simulink model "HRTIM_main"  (R2023b)
settings: Solver=ode3  StartTime=0.0  StopTime=120e-6  RelTol=1e-3
undefined symbols (not defined in the file): HRTIM_SETB1R_REG_VAL, HRTIM_SETB2R_REG_VAL, HRTIM_SETC1R_REG_VAL, HRTIM_SETC2R_REG_VAL, HRTIM_SL
libraries: dspswit3 x8, simulink x6, simulink_extras x4, hdlsllib x4
(part 2 of 2)

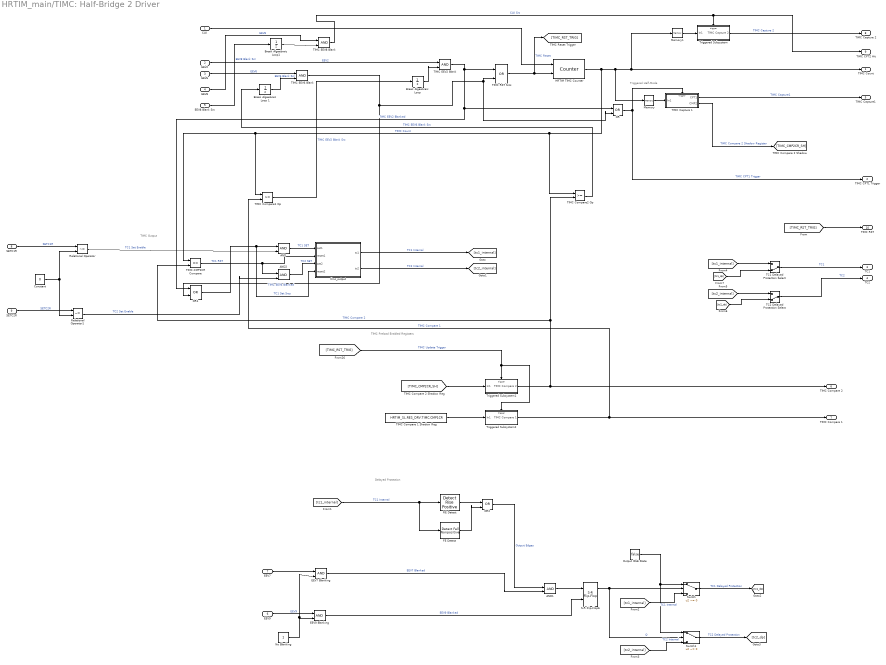
== system HRTIM_main/TIMC: Half-Bridge 2 Driver ==
  note: TIMC Preload Enabled Registers
  note: Triggered Half-Mode
  note: TIMC Output
  note: Delayed Protection
  CLK : Inport
  EEV2 : Inport  Port=2
  EEV6 : Inport  Port=3
  EEV8 : Inport  Port=4
  EEV8 Blank Src : Inport  Port=5
  EEV9 : Inport  Port=6
  EEV7 : Inport  Port=7
  SETC1R : Inport  Port=8
  SETC2R : Inport  Port=9
  AND : Logic  IconShape=distinctive  AllPortsSameDT=off  OutDataTypeStr=boolean
  AND1 : Logic  IconShape=distinctive  AllPortsSameDT=off  OutDataTypeStr=boolean
  AND2 : Logic  IconShape=distinctive  AllPortsSameDT=off  OutDataTypeStr=boolean
  Break Algaebraic Loop : UnitDelay  SampleTime=-1  HasFrameUpgradeWarning=on
  Break Algaebraic Loop 1 : UnitDelay  SampleTime=-1  HasFrameUpgradeWarning=on
  Break Algaebraic Loop1 : UnitDelay  SampleTime=-1  HasFrameUpgradeWarning=on
  Constant : Constant  Value=0  OutDataTypeStr=uint32
  EEV7 Blanking : Logic  IconShape=distinctive  AllPortsSameDT=off  OutDataTypeStr=boolean
  EEV9 Blanking : Logic  IconShape=distinctive  AllPortsSameDT=off  OutDataTypeStr=boolean
  FE Detect : simulink/Logic and Bit Operations/Detect Fall Nonpositive  vinit=0  OutDataTypeStr=boolean
  HRTIM TIMC Counter : dspswit3/Counter  Direction=Up  CountEvent=Rising edge  CounterSize=16 bits  MaxCount=HRTIM_SL.HRTIM_TIMx_FS  InitialCount=0  Output=Count  HitValue=32  ResetInput=on  SamplesPerFrame=1  Ts=1  CntDtype=uint16  HitDtype=Logical
  Memory : Memory  InheritSampleTime=on
  Memory1 : Memory
  No Blanking : Constant
  OR : Logic  Operator=OR  IconShape=distinctive  AllPortsSameDT=off  OutDataTypeStr=boolean
  OR1 : Logic  Operator=OR  IconShape=distinctive  AllPortsSameDT=off  OutDataTypeStr=boolean
  OR2 : Logic  Operator=OR  IconShape=distinctive  AllPortsSameDT=off  OutDataTypeStr=boolean
  Output IDLE State : Constant  Value=false  OutDataTypeStr=boolean
  RE Detect : hdlsllib/Logic and Bit Operations/Detect Rise Positive  vinit=0  OutDataTypeStr=boolean
  Relational Operator : RelationalOperator  Operator=~=  OutDataTypeStr=boolean  RndMeth=Simplest  InputSameDT=off
  Relational Operator1 : RelationalOperator  Operator=~=  OutDataTypeStr=boolean  RndMeth=Simplest  InputSameDT=off
  S-R Flip-Flop6 : simulink_extras/Flip Flops/S-R Flip-Flop  initial_condition=0
  Switch : Switch  Criteria=u2 ~= 0  SaturateOnIntegerOverflow=off  InputSameDT=off
  Switch1 : Switch  Criteria=u2 ~= 0  SaturateOnIntegerOverflow=off  InputSameDT=off
  TC1 Delayed Protection Select : ManualSwitch  CurrentSetting=0
  TC2 Delayed Protection Select : ManualSwitch  CurrentSetting=0
  TIMC Capture 1 : Subsystem  TreatAsAtomicUnit=on
  TIMC Compare 1 Shadow Reg : Constant  Value=HRTIM_SL.RES_DRV.TIMC.CMP1CR
  TIMC Compare1 Op : RelationalOperator  OutDataTypeStr=boolean  RndMeth=Simplest  InputSameDT=off
  TIMC Compare2 Op : RelationalOperator  OutDataTypeStr=boolean  RndMeth=Simplest  InputSameDT=off
  TIMC EEV2 Blank : Logic  IconShape=distinctive  AllPortsSameDT=off  OutDataTypeStr=boolean
  TIMC EEV6 Blank : Logic  IconShape=distinctive  AllPortsSameDT=off  OutDataTypeStr=boolean
  TIMC EEV8 Blank : Logic  IconShape=distinctive  AllPortsSameDT=off  OutDataTypeStr=boolean
  TIMC RST Srcs : Logic  Operator=OR  IconShape=distinctive  AllPortsSameDT=off  OutDataTypeStr=boolean
  TIMC.CMP2CR Compare : RelationalOperator  Operator===  OutDataTypeStr=boolean  RndMeth=Simplest  InputSameDT=off
  Triggered Subsystem : Subsystem  TreatAsAtomicUnit=on
  Triggered Subsystem1 : Subsystem  TreatAsAtomicUnit=on
  Triggered Subsystem2 : Subsystem  TreatAsAtomicUnit=on
  timc_output : MATLAB Function  TreatAsAtomicUnit=on
  TIMC Count : Outport
  TIMC CPT1 Trigger : Outport  Port=2
  TC1 : Outport  Port=3
  TC2 : Outport  Port=4
  TIMC Capture1 : Outport  Port=5
  TIMC Compare 2 : Outport  Port=6
  TIMC Compare 1 : Outport  Port=7
  TIMC Capture 2 : Outport  Port=8
  TIMC CPT2 Hit : Outport  Port=9
  TIMC RST : Outport  Port=10
  wires:
  TIMC EEV6 Blank/1 -> OR1/2, TIMC RST Srcs/2, OR/2  "TIMC EEV6 Blanked"
  [TIMC_CMP2CR_SH] -> Triggered Subsystem1/1(In1)
  HRTIM TIMC Counter/1 -> Memory1/1, TIMC Count/1, Memory/1, TIMC.CMP2CR Compare/1, TIMC Compare1 Op/1, TIMC Compare2 Op/1  "TIMC Count"
  TIMC Compare1 Op/1 -> Break Algaebraic Loop/1  "TIMC EEV2 Blank Src"
  TIMC Capture 1/2(CMP2) -> [TIMC_CMP2CR_SH]  "TIMC Compare 2 Shadow Register"
  TIMC EEV2 Blank/1 -> OR1/1, OR/1, TIMC RST Srcs/1  "TIMC EEV2 Blanked"
  [TIMC_RST_TRIG] -> Triggered Subsystem2/Trigger, Triggered Subsystem1/Trigger  "TIMC Update Trigger"
  TIMC RST Srcs/1 -> HRTIM TIMC Counter/2, [TIMC_RST_TRIG]  "TIMC Reset"
  Memory/1 -> TIMC Capture 1/1(In1)
  Break Algaebraic Loop 1/1 -> TIMC EEV6 Blank/2  "EEV6 Blank Src"
  OR/1 -> TIMC CPT1 Trigger/1, TIMC Capture 1/Trigger  "TIMC CPT1 Trigger"
  Break Algaebraic Loop/1 -> TIMC EEV2 Blank/2
  Triggered Subsystem1/1(TIMC Compare 2) -> TIMC Compare2 Op/2, TIMC.CMP2CR Compare/2, TIMC Compare 2/1  "TIMC Compare 2"
  EEV2/1 -> TIMC EEV2 Blank/1  "EEV2"
  TIMC Compare2 Op/1 -> Break Algaebraic Loop 1/1  "TIMC EEV6 Blank Src"
  Triggered Subsystem2/1(TIMC Compare 1) -> TIMC Compare1 Op/2, TIMC Compare 1/1  "TIMC Compare 1"
  TIMC Compare 1 Shadow Reg/1 -> Triggered Subsystem2/1(In1)
  TIMC Capture 1/1(CPT1) -> TIMC Capture1/1  "TIMC Capture1"
  CLK/1 -> HRTIM TIMC Counter/1
  EEV6/1 -> TIMC EEV6 Blank/1  "EEV6"
  TIMC.CMP2CR Compare/1 -> timc_output/2(reset1), AND2/1  "TC1 RST"
  Triggered Subsystem/1(TIMC Capture 2) -> TIMC Capture 2/1  "TIMC Capture 2"
  EEV8/1 -> TIMC EEV8 Blank/1  "EEV8"
  EEV8 Blank Src/1 -> Break Algaebraic Loop1/1  "EEV8 Blank Src"
  TIMC EEV8 Blank/1 -> Triggered Subsystem/Trigger, TIMC CPT2 Hit/1  "CLK Src"
  Memory1/1 -> Triggered Subsystem/1(In1)
  Break Algaebraic Loop1/1 -> TIMC EEV8 Blank/2
  timc_output/1(tc1) -> [tc1_internal]  "TC1 Internal"
  timc_output/2(tc2) -> [tc2_internal]  "TC2 Internal"
  TC1 Delayed Protection Select/1 -> TC1/1  "TC1"
  [tc1_dp] -> TC1 Delayed Protection Select/2
  [tc2_internal] -> TC2 Delayed Protection Select/1
  [tc2_dp] -> TC2 Delayed Protection Select/2
  TC2 Delayed Protection Select/1 -> TC2/1  "TC2"
  [tc1_internal] -> TC1 Delayed Protection Select/1
  Switch1/1 -> [tc2_dp]  "TC2 Delayed Protection"
  AND1/1 -> S-R Flip-Flop6/1
  [tc2_internal] -> Switch1/3  "TC2 Internal"
  EEV9/1 -> EEV9 Blanking/1  "EEV9"
  [tc1_internal] -> FE Detect/1, RE Detect/1  "TC1 Internal"
  Switch/1 -> [tc1_dp]  "TC1 Delayed Protection"
  RE Detect/1 -> OR2/1
  FE Detect/1 -> OR2/2
  OR2/1 -> AND1/1  "Output Edges"
  EEV7/1 -> EEV7 Blanking/1
  No Blanking/1 -> EEV9 Blanking/2, EEV7 Blanking/2
  EEV7 Blanking/1 -> AND1/2  "EEV7 Blanked"
  [tc1_internal] -> Switch/3  "TC1 Internal"
  S-R Flip-Flop6/1 -> Switch/2, Switch1/2  "Q"
  Output IDLE State/1 -> Switch/1, Switch1/1
  EEV9 Blanking/1 -> S-R Flip-Flop6/2  "EEV9 Blanked"
  [TIMC_RST_TRIG] -> TIMC RST/1
  SETC1R/1 -> Relational Operator/1  "SETC1R"
  Constant/1 -> Relational Operator/2, Relational Operator1/2
  OR1/1 -> AND/1, timc_output/4(reset2)  "TC1 Set Srcs"
  AND/1 -> timc_output/1(set1)  "TC1 SET"
  Relational Operator/1 -> AND/2  "TC1 Set Enable"
  AND2/1 -> timc_output/3(set2)  "TC2 SET"
  Relational Operator1/1 -> AND2/2  "TC2 Set Enable"
  SETC2R/1 -> Relational Operator1/1  "SETC2R"

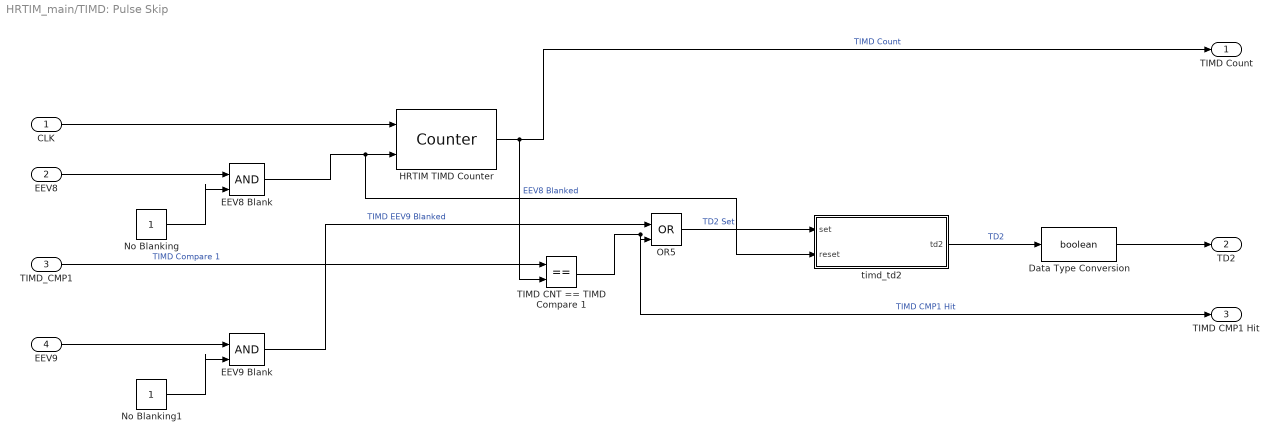
== system HRTIM_main/TIMD: Pulse Skip ==
  CLK : Inport
  EEV8 : Inport  Port=2
  TIMD_CMP1 : Inport  Port=3
  EEV9 : Inport  Port=4
  Data Type Conversion : DataTypeConversion  OutDataTypeStr=boolean  SaturateOnIntegerOverflow=off  RndMeth=Floor
  EEV8 Blank : Logic  IconShape=distinctive  AllPortsSameDT=off  OutDataTypeStr=boolean
  EEV9 Blank : Logic  IconShape=distinctive  AllPortsSameDT=off  OutDataTypeStr=boolean
  HRTIM TIMD Counter : dspswit3/Counter  Direction=Up  CountEvent=Rising edge  CounterSize=16 bits  MaxCount=HRTIM_SL.HRTIM_TIMx_FS  InitialCount=0  Output=Count  HitValue=32  ResetInput=on  SamplesPerFrame=1  Ts=1  CntDtype=uint16  HitDtype=Logical
  No Blanking : Constant
  No Blanking1 : Constant
  OR5 : Logic  Operator=OR  IconShape=distinctive  AllPortsSameDT=off  OutDataTypeStr=boolean
  TIMD CNT == TIMD Compare 1 : RelationalOperator  Operator===  OutDataTypeStr=boolean  RndMeth=Simplest  InputSameDT=off
  timd_td2 : MATLAB Function  TreatAsAtomicUnit=on
  TIMD Count : Outport
  TD2 : Outport  Port=2
  "TIMD CMP1 Hit " : Outport  Port=3
  wires:
  No Blanking/1 -> EEV8 Blank/2
  HRTIM TIMD Counter/1 -> TIMD Count/1, TIMD CNT == TIMD Compare 1/2  "TIMD Count"
  EEV9/1 -> EEV9 Blank/1
  timd_td2/1(td2) -> Data Type Conversion/1  "TD2"
  No Blanking1/1 -> EEV9 Blank/2
  EEV8 Blank/1 -> HRTIM TIMD Counter/2, timd_td2/2(reset)  "EEV8 Blanked"
  TIMD CNT == TIMD Compare 1/1 -> "TIMD CMP1 Hit "/1, OR5/2  "TIMD CMP1 Hit"
  OR5/1 -> timd_td2/1(set)  "TD2 Set"
  CLK/1 -> HRTIM TIMD Counter/1
  EEV9 Blank/1 -> OR5/1  "TIMD EEV9 Blanked"
  EEV8/1 -> EEV8 Blank/1
  TIMD_CMP1/1 -> TIMD CNT == TIMD Compare 1/1  "TIMD Compare 1"
  Data Type Conversion/1 -> TD2/1

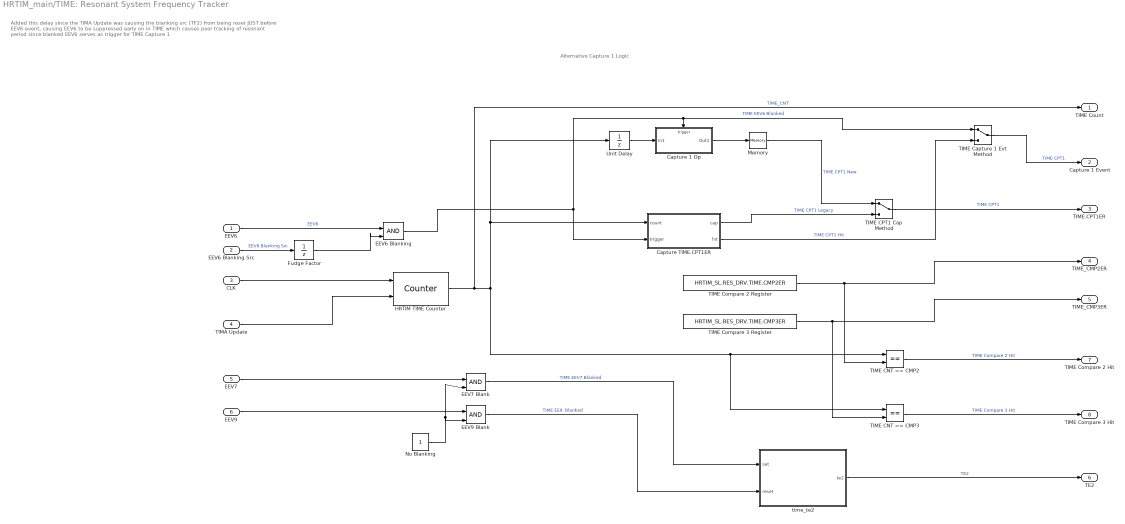
== system HRTIM_main/TIME: Resonant System Frequency Tracker ==
  note: Added this delay since the TIMA Update was causing the blanking src (TF2) from being reset JUST before EEV6 event, causing EEV6 to be suppressed early on in TIME which causes poor tracking of resonant period since blanked EEV6 serves as trigger for TIME Capture 1
  note: Alternative Capture 1 Logic
  EEV6 : Inport
  EEV6 Blanking Src : Inport  Port=2
  CLK : Inport  Port=3
  TIMA Update : Inport  Port=4
  EEV7 : Inport  Port=5
  EEV9 : Inport  Port=6
  Capture 1 Op : Subsystem  TreatAsAtomicUnit=on
  Capture TIME.CPT1ER : MATLAB Function  TreatAsAtomicUnit=on
  EEV6 Blanking : Logic  IconShape=distinctive  AllPortsSameDT=off  OutDataTypeStr=boolean
  EEV7 Blank : Logic  IconShape=distinctive  AllPortsSameDT=off  OutDataTypeStr=boolean
  EEV9 Blank : Logic  IconShape=distinctive  AllPortsSameDT=off  OutDataTypeStr=boolean
  Fudge Factor : UnitDelay  SampleTime=-1  HasFrameUpgradeWarning=on
  HRTIM TIME Counter : dspswit3/Counter  Direction=Up  CountEvent=Rising edge  CounterSize=16 bits  MaxCount=HRTIM_SL.HRTIM_TIMx_FS  InitialCount=0  Output=Count  HitValue=32  ResetInput=on  SamplesPerFrame=1  Ts=1  CntDtype=uint16  HitDtype=Logical
  Memory : Memory
  No Blanking : Constant
  TIME CNT == CMP2 : RelationalOperator  Operator===  OutDataTypeStr=boolean  RndMeth=Simplest  InputSameDT=off
  TIME CNT == CMP3 : RelationalOperator  Operator===  OutDataTypeStr=boolean  RndMeth=Simplest  InputSameDT=off
  TIME CPT1 Cap Method : ManualSwitch
  TIME Capture 1 Evt Method : ManualSwitch
  TIME Compare 2 Register : Constant  Value=HRTIM_SL.RES_DRV.TIME.CMP2ER
  TIME Compare 3 Register : Constant  Value=HRTIM_SL.RES_DRV.TIME.CMP3ER
  Unit Delay : UnitDelay  SampleTime=-1  HasFrameUpgradeWarning=on
  time_te2 : MATLAB Function  TreatAsAtomicUnit=on
  TIME Count : Outport
  Capture 1 Event : Outport  Port=2
  TIME.CPT1ER : Outport  Port=3
  TIME_CMP2ER : Outport  Port=4
  TIME_CMP3ER : Outport  Port=5
  TE2 : Outport  Port=6
  TIME Compare 2 Hit : Outport  Port=7
  TIME Compare 3 Hit : Outport  Port=8
  wires:
  EEV6 Blanking/1 -> Capture 1 Op/Trigger, TIME Capture 1 Evt Method/1, Capture TIME.CPT1ER/2(trigger)  "TIME EEV6 Blanked"
  EEV6/1 -> EEV6 Blanking/1  "EEV6"
  Capture TIME.CPT1ER/1(cap) -> TIME CPT1 Cap Method/2  "TIME CPT1 Legacy"
  time_te2/1(te2) -> TE2/1  "TE2"
  EEV6 Blanking Src/1 -> Fudge Factor/1  "EEV6 Blanking Src"
  TIME Compare 3 Register/1 -> TIME_CMP3ER/1, TIME CNT == CMP3/2
  HRTIM TIME Counter/1 -> TIME Count/1, TIME CNT == CMP2/1, TIME CNT == CMP3/1, Unit Delay/1, Capture TIME.CPT1ER/1(count)  "TIME_CNT"
  CLK/1 -> HRTIM TIME Counter/1
  TIME Compare 2 Register/1 -> TIME_CMP2ER/1, TIME CNT == CMP2/2
  TIMA Update/1 -> HRTIM TIME Counter/2
  EEV7/1 -> EEV7 Blank/1
  EEV7 Blank/1 -> time_te2/1(set)  "TIME EEV7 Blanked"
  EEV9/1 -> EEV9 Blank/1
  EEV9 Blank/1 -> time_te2/2(reset)  "TIME EE9  Blanked"
  No Blanking/1 -> EEV9 Blank/2, EEV7 Blank/2
  Capture 1 Op/1(Out1) -> Memory/1
  Fudge Factor/1 -> EEV6 Blanking/2
  TIME CPT1 Cap Method/1 -> TIME.CPT1ER/1  "TIME CPT1"
  Memory/1 -> TIME CPT1 Cap Method/1  "TIME CPT1 New"
  TIME Capture 1 Evt Method/1 -> Capture 1 Event/1  "TIME CPT1"
  Capture TIME.CPT1ER/2(hit) -> TIME Capture 1 Evt Method/2  "TIME CPT1 Hit"
  Unit Delay/1 -> Capture 1 Op/1(In1)
  TIME CNT == CMP2/1 -> TIME Compare 2 Hit/1  "TIME Compare 2 Hit"
  TIME CNT == CMP3/1 -> TIME Compare 3 Hit/1  "TIME Compare 3 Hit"

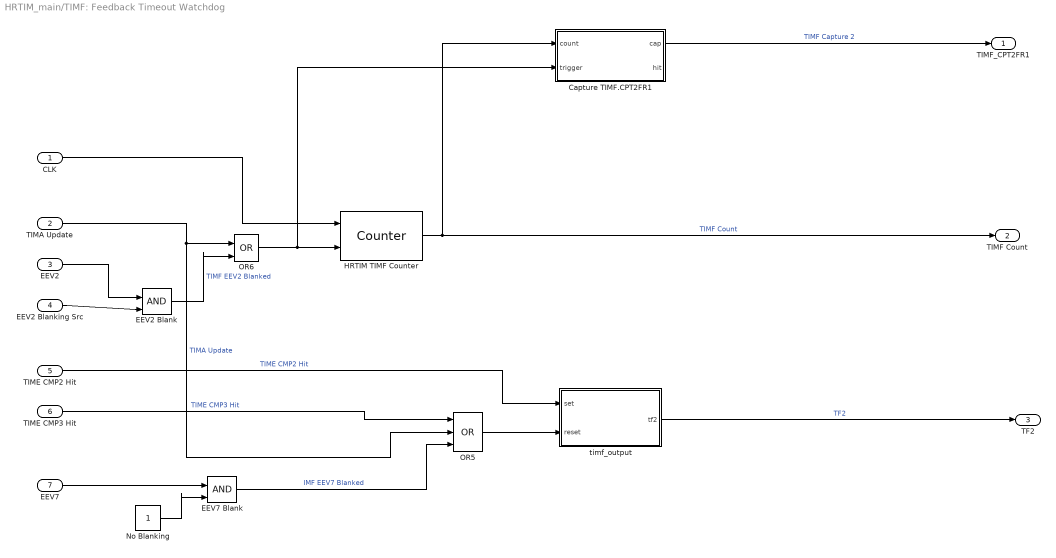
== system HRTIM_main/TIMF: Feedback Timeout Watchdog ==
  CLK : Inport
  TIMA Update : Inport  Port=2
  EEV2 : Inport  Port=3
  EEV2 Blanking Src : Inport  Port=4
  TIME CMP2 Hit : Inport  Port=5
  TIME CMP3 Hit : Inport  Port=6
  EEV7 : Inport  Port=7
  Capture TIMF.CPT2FR1 : MATLAB Function  TreatAsAtomicUnit=on
  EEV2 Blank : Logic  IconShape=distinctive  AllPortsSameDT=off  OutDataTypeStr=boolean
  EEV7 Blank : Logic  IconShape=distinctive  AllPortsSameDT=off  OutDataTypeStr=boolean
  HRTIM TIMF Counter : dspswit3/Counter  Direction=Up  CountEvent=Rising edge  CounterSize=16 bits  MaxCount=HRTIM_SL.HRTIM_TIMx_FS  InitialCount=0  Output=Count  HitValue=32  ResetInput=on  SamplesPerFrame=1  Ts=1  CntDtype=uint16  HitDtype=Logical
  No Blanking : Constant
  OR5 : Logic  Operator=OR  Inputs=3  IconShape=distinctive  AllPortsSameDT=off  OutDataTypeStr=boolean
  OR6 : Logic  Operator=OR  IconShape=distinctive  AllPortsSameDT=off  OutDataTypeStr=boolean
  timf_output : MATLAB Function  TreatAsAtomicUnit=on
  TIMF_CPT2FR1 : Outport
  TIMF Count : Outport  Port=2
  TF2 : Outport  Port=3
  wires:
  TIMA Update/1 -> OR5/2, OR6/1  "TIMA Update"
  HRTIM TIMF Counter/1 -> TIMF Count/1, Capture TIMF.CPT2FR1/1(count)  "TIMF Count"
  EEV2 Blank/1 -> OR6/2  "TIMF EEV2 Blanked"
  EEV7 Blank/1 -> OR5/3  "IMF EEV7 Blanked"
  EEV2/1 -> EEV2 Blank/1
  Capture TIMF.CPT2FR1/1(cap) -> TIMF_CPT2FR1/1  "TIMF Capture 2"
  OR6/1 -> Capture TIMF.CPT2FR1/2(trigger), HRTIM TIMF Counter/2
  No Blanking/1 -> EEV7 Blank/2
  OR5/1 -> timf_output/2(reset)
  EEV2 Blanking Src/1 -> EEV2 Blank/2
  timf_output/1(tf2) -> TF2/1  "TF2"
  TIME CMP3 Hit/1 -> OR5/1  "TIME CMP3 Hit"
  TIME CMP2 Hit/1 -> timf_output/1(set)  "TIME CMP2 Hit"
  CLK/1 -> HRTIM TIMF Counter/1
  EEV7/1 -> EEV7 Blank/1

== system HRTIM_main/Update TIMB SETBxR Active Registers ==
  In1 : Inport
  In2 : Inport  Port=2
  Trigger : TriggerPort  VariantControl=(inherit)
  Out1 : Outport
  Out2 : Outport  Port=2
  wires:
  In1/1 -> Out1/1
  In2/1 -> Out2/1

== system HRTIM_main/Update TIMB SETCxR Active Registers ==
  In1 : Inport
  In2 : Inport  Port=2
  Trigger : TriggerPort  VariantControl=(inherit)
  Out1 : Outport
  Out2 : Outport  Port=2
  wires:
  In1/1 -> Out1/1
  In2/1 -> Out2/1

== system HRTIM_main/out_reset_toggle ==
  note: This is artificially prolonging the delay so that the alternating states of the SETxyR registers persist long enough for the down stream TIMB and TIMC update events to actually propagate the new state from the shadow registers to the active registers (before they toggle back to the old state).
  Trigger : TriggerPort  VariantControl=(inherit)
  Delay : Delay  DelayLength=4
  NOT2 : Logic  Operator=NOT  IconShape=distinctive  AllPortsSameDT=off  OutDataTypeStr=boolean
  Out1 : Outport
  wires:
  Delay/1 -> NOT2/1
  NOT2/1 -> Delay/1, Out1/1

== system HRTIM_main/TIM2: Start Freq Seed + Lead Time Inject/TIM2 ARR Preload Op ==
  In1 : Inport
  Trigger : TriggerPort  VariantControl=(inherit)
  TIM2 ARR : Outport  InitialOutput=HRTIM_SL.RES_DRV.TIM2.ARR
  wires:
  In1/1 -> TIM2 ARR/1

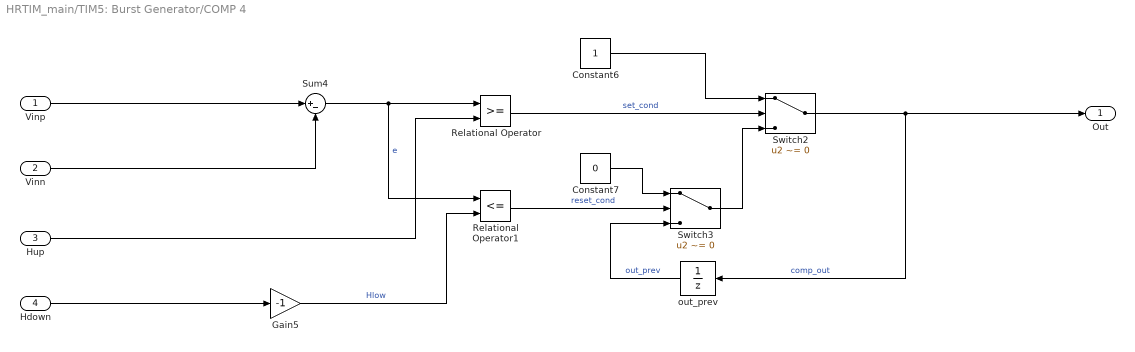
== system HRTIM_main/TIM5: Burst Generator/COMP 4 ==
  Vinp : Inport
  Vinn : Inport  Port=2
  Hup : Inport  Port=3
  Hdown : Inport  Port=4
  Constant6 : Constant
  Constant7 : Constant  Value=0
  Gain5 : Gain  Gain=-1
  Relational Operator : RelationalOperator  OutDataTypeStr=boolean  RndMeth=Simplest  InputSameDT=off
  Relational Operator1 : RelationalOperator  Operator=<=  OutDataTypeStr=boolean  RndMeth=Simplest  InputSameDT=off
  Sum4 : Sum  Inputs=|+-
  Switch2 : Switch  Criteria=u2 ~= 0  SaturateOnIntegerOverflow=off  InputSameDT=off
  Switch3 : Switch  Criteria=u2 ~= 0  SaturateOnIntegerOverflow=off  InputSameDT=off
  out_prev : UnitDelay  SampleTime=-1  HasFrameUpgradeWarning=on
  Out : Outport
  wires:
  Sum4/1 -> Relational Operator/1, Relational Operator1/1  "e"
  Relational Operator/1 -> Switch2/2  "set_cond"
  Switch2/1 -> Out/1, out_prev/1  "comp_out"
  Relational Operator1/1 -> Switch3/2  "reset_cond"
  Vinn/1 -> Sum4/2
  Gain5/1 -> Relational Operator1/2  "Hlow"
  Constant6/1 -> Switch2/1
  out_prev/1 -> Switch3/3  "out_prev"
  Hup/1 -> Relational Operator/2
  Constant7/1 -> Switch3/1
  Vinp/1 -> Sum4/1
  Switch3/1 -> Switch2/3
  Hdown/1 -> Gain5/1

== system HRTIM_main/TIMA: Master reference/Triggered Subsystem1 ==
  In1 : Inport
  Trigger : TriggerPort  VariantControl=(inherit)
  TIMA Compare 2 : Outport
  wires:
  In1/1 -> TIMA Compare 2/1

== system HRTIM_main/TIMA: Master reference/Triggered Subsystem2 ==
  In1 : Inport
  Trigger : TriggerPort  VariantControl=(inherit)
  TIMA Compare 1 : Outport
  wires:
  In1/1 -> TIMA Compare 1/1

== system HRTIM_main/TIMB: Half-Bridge 1 Driver/TIMB Capture 1 ==
  In1 : Inport
  Trigger : TriggerPort  VariantControl=(inherit)  InitialTriggerSignalState=zero
  Bit Shift : hdlsllib/Logic and Bit Operations/Bit Shift  mode=Shift Right Arithmetic  N=1
  CPT1 : Outport
  CMP2 : Outport  Port=2
  wires:
  Bit Shift/1 -> CMP2/1
  In1/1 -> Bit Shift/1, CPT1/1

== system HRTIM_main/TIMB: Half-Bridge 1 Driver/Triggered Subsystem ==
  In1 : Inport
  Trigger : TriggerPort  VariantControl=(inherit)
  TIMB Capture 2 : Outport
  wires:
  In1/1 -> TIMB Capture 2/1

== system HRTIM_main/TIMB: Half-Bridge 1 Driver/Triggered Subsystem1 ==
  In1 : Inport
  Trigger : TriggerPort  VariantControl=(inherit)
  TIMB Compare 2 : Outport
  wires:
  In1/1 -> TIMB Compare 2/1

== system HRTIM_main/TIMB: Half-Bridge 1 Driver/Triggered Subsystem2 ==
  In1 : Inport
  Trigger : TriggerPort  VariantControl=(inherit)
  TIMB Compare 1 : Outport
  wires:
  In1/1 -> TIMB Compare 1/1

== system HRTIM_main/TIMC: Half-Bridge 2 Driver/TIMC Capture 1 ==
  In1 : Inport
  Trigger : TriggerPort  VariantControl=(inherit)  InitialTriggerSignalState=zero
  Bit Shift : hdlsllib/Logic and Bit Operations/Bit Shift  mode=Shift Right Arithmetic  N=1
  CPT1 : Outport
  CMP2 : Outport  Port=2
  wires:
  Bit Shift/1 -> CMP2/1
  In1/1 -> Bit Shift/1, CPT1/1

== system HRTIM_main/TIMC: Half-Bridge 2 Driver/Triggered Subsystem ==
  In1 : Inport
  Trigger : TriggerPort  VariantControl=(inherit)
  TIMC Capture 2 : Outport
  wires:
  In1/1 -> TIMC Capture 2/1

== system HRTIM_main/TIMC: Half-Bridge 2 Driver/Triggered Subsystem1 ==
  In1 : Inport
  Trigger : TriggerPort  VariantControl=(inherit)
  TIMC Compare 2 : Outport
  wires:
  In1/1 -> TIMC Compare 2/1

== system HRTIM_main/TIMC: Half-Bridge 2 Driver/Triggered Subsystem2 ==
  In1 : Inport
  Trigger : TriggerPort  VariantControl=(inherit)
  TIMC Compare 1 : Outport
  wires:
  In1/1 -> TIMC Compare 1/1

== system HRTIM_main/TIME: Resonant System Frequency Tracker/Capture 1 Op ==
  In1 : Inport
  Trigger : TriggerPort  VariantControl=(inherit)
  Out1 : Outport  InitialOutput=0
  wires:
  In1/1 -> Out1/1

== matlab function HRTIM_main/TIMB: Half-Bridge 1 Driver/timb_output ==
  data: set1 input; tb1 output boolean; reset1 input; tb2 output; set2 input; reset2 input
function [tb1,tb2] = timb_output(set1,reset1,set2,reset2)

persistent set1_prev;
persistent reset1_prev;

persistent set2_prev;
persistent reset2_prev;

persistent tb1_prev;
persistent tb2_prev;

% Init persistent var on first iter
if isempty(set1_prev)
    set1_prev = set1; 
end

if isempty(reset1_prev)
    reset1_prev = reset1; 
end

if isempty(set2_prev)
    set2_prev = set2; 
end

if isempty(reset2_prev)
    reset2_prev = reset2; 
end

if isempty(tb1_prev)
    tb1_prev = false; 
end

if isempty(tb2_prev)
    tb2_prev = false; 
end

tb1 = tb1_prev;
tb2 = tb2_prev;

% Check for rising edge on SET input
set1_re  = (set1 > 0) && (set1_prev <= 0); 
% Check for rising edge on RESET input
reset1_re  = (reset1 > 0) && (reset1_prev <= 0);

set2_re  = (set2 > 0) && (set2_prev <= 0); 
% Check for rising edge on RESET input
reset2_re  = (reset2 > 0) && (reset2_prev <= 0);

if set1_re
    tb1 = true;
end

if reset1_re
    tb1 = false;
end

if set2_re
    tb2 = true;
end

if reset2_re
    tb2 = false;
end


% Update persistent var for next iteration
set1_prev = set1;
reset1_prev = reset1;
tb1_prev = tb1;

set2_prev = set2;
reset2_prev = reset2;
tb2_prev = tb2;

end

== matlab function HRTIM_main/TIMC: Half-Bridge 2 Driver/timc_output ==
  data: set1 input; tc1 output boolean; reset1 input; tc2 output; set2 input; reset2 input
function [tc1,tc2] = timb_output(set1,reset1,set2,reset2)

persistent set1_prev;
persistent reset1_prev;

persistent set2_prev;
persistent reset2_prev;

persistent tc1_prev;
persistent tc2_prev;

% Init persistent var on first iter
if isempty(set1_prev)
    set1_prev = set1; 
end

if isempty(reset1_prev)
    reset1_prev = reset1; 
end

if isempty(set2_prev)
    set2_prev = set2; 
end

if isempty(reset2_prev)
    reset2_prev = reset2; 
end

if isempty(tc1_prev)
    tc1_prev = false; 
end

if isempty(tc2_prev)
    tc2_prev = false; 
end

tc1 = tc1_prev;
tc2 = tc2_prev;

% Check for rising edge on SET input
set1_re  = (set1 > 0) && (set1_prev <= 0); 
% Check for rising edge on RESET input
reset1_re  = (reset1 > 0) && (reset1_prev <= 0);

set2_re  = (set2 > 0) && (set2_prev <= 0); 
% Check for rising edge on RESET input
reset2_re  = (reset2 > 0) && (reset2_prev <= 0);

if set1_re
    tc1 = true;
end

if reset1_re
    tc1 = false;
end

if set2_re
    tc2 = true;
end

if reset2_re
    tc2 = false;
end


% Update persistent var for next iteration
set1_prev = set1;
reset1_prev = reset1;
tc1_prev = tc1;

set2_prev = set2;
reset2_prev = reset2;
tc2_prev = tc2;

end

== matlab function HRTIM_main/TIMA: Master reference/eev9_latch ==
  data: eev input; eev_blanked output; blank_src input
function eev_blanked = eev_latch(eev,blank_src)

% This block mimics the latch behavior for EEV event blanking
% for each TIM within the HRTIM. If EEV occurs when the blanking signal is
% low (i.e. mask/suppress event) then latch the event so that when the blanking
% signal goes high (i.e. unmask event) the latched, post-poned signal is
% propagated to the output

persistent eev_prev;
persistent eev_re_latched;

% Init persistent var on first iter
if isempty(eev_prev)
    eev_prev = eev; 
end

if isempty(eev_re_latched)
    eev_re_latched = false; 
end

eev_blanked = false;

% Detect rising edge of EEV input
eev_re  = (eev > 0) && (eev_prev <= 0); 

% If EEV occurred when blanking is high (unmasked): allow EEV to propagate
% to output immediately
if eev_re == true && blank_src == true
   eev_blanked = true;
end

% If EEV occurred when blanking is low (masked): latch EEV, and postpone to
% next rising edge of blank signal
if eev_re == true && blank_src == false
    eev_re_latched = true;
end

% If EEV was previously latched, propagate the post-poned event to the
% output at the this blanking src rising edge
if eev_re_latched == true && blank_src == true
    eev_blanked = true;
    eev_re_latched = false;
end

% Update persistent var for next iteration
eev_prev = eev;

== matlab function HRTIM_main/TIME: Resonant System Frequency Tracker/Capture TIME.CPT1ER ==
  data: count input; cap output; trigger input; hit output
function [cap,hit] = capture_reg(count,trigger)

% hit generates positive pulse when capture occurs

persistent count_prev;
persistent trigger_prev;

persistent cap_reg;

% Init persistent variables
if isempty(count_prev)
    count_prev = count; 
end

if isempty(trigger_prev)
    trigger_prev = trigger; 
end

if isempty(cap_reg)
    cap_reg = uint16(0); 
end

hit = 0;

% Trigger rising edge detect
trigger_re  = (trigger > 0) && (trigger_prev <= 0); 

% Capture register on rising edge of trigger
% Use previous count since we are 1 sample behind
if trigger_re
    cap_reg = count_prev;
    hit = 1;
end

% Update persistent var
count_prev = count;
trigger_prev = trigger;

cap = cap_reg;

== matlab function HRTIM_main/TIME: Resonant System Frequency Tracker/time_te2 ==
  data: te2 output; set input; reset input
function te2 = time_te2(set,reset)

persistent set_prev;
persistent reset_prev;
persistent te2_prev;

% Init persistent var on first iter
if isempty(set_prev)
    set_prev = set; 
end

if isempty(reset_prev)
    reset_prev = reset; 
end

if isempty(te2_prev)
    te2_prev = 0; 
end

te2 = te2_prev;

% Check for rising edge on SET input
set_re  = (set > 0) && (set_prev <= 0); 
% Check for rising edge on RESET input
reset_re  = (reset > 0) && (reset_prev <= 0);

if set_re
    te2 = 1;
end

if reset_re
    te2 = 0;
end

% Update persistent var for next iteration
set_prev = set;
reset_prev = reset;
te2_prev = te2;

end

== matlab function HRTIM_main/TIM5: Burst Generator/gen_eev7_eev9 ==
  data: comp4_out input; eev7 output; eev9 output
function [eev7,eev9] = gen_eev7_eev9(comp4_out)

persistent comp4_out_prev;
persistent eev7_prev;
persistent eev9_prev;

% Init persistent var on first iter
if isempty(comp4_out_prev)
    comp4_out_prev = comp4_out; 
end

if isempty(eev7_prev)
    eev7_prev = 0; 
end

if isempty(eev9_prev)
    eev9_prev = 0; 
end

eev7 = eev7_prev;
eev9 = eev9_prev;

% Check for rising edge on SET input
comp4_re  = (comp4_out > 0) && (comp4_out_prev <= 0); 

if comp4_re
    eev9 = 1;
else
    eev9 = 0;
end

% Check for COMP4 low level
if comp4_out == 0
    eev7 = 1;
else
    eev7 = 0;
end

% Update persistent var for next iteration
comp4_out_prev = comp4_out;
eev7_prev = eev7;
eev9_prev = eev9;

end

== matlab function HRTIM_main/TIMA: Master reference/gen_tima_update ==
  data: count input; update output; reset input
function update  = gen_tima_update(count,reset)

persistent count_prev;
persistent reset_prev;
persistent update_prev;

% Init persistent var on first iter
if isempty(count_prev)
    count_prev = count; 
end

if isempty(reset_prev)
    reset_prev = reset; 
end

if isempty(update_prev)
    update_prev = 0; 
end

update = update_prev;

% Check for rising edge on SET input
reset_re  = (reset > 0) && (reset_prev <= 0); 
counter_rollover  = (count == 0) && (count_prev > 0);

if reset_re || counter_rollover
    update = 1;
else
    update = 0;
end

% Update persistent var for next iteration
update_prev = update;
count_prev = count;
reset_prev = reset;

end

== matlab function HRTIM_main/TIMA: Master reference/tima_ta2 ==
  data: set input; ta2 output; reset input
function ta2 = tima_ta2(set,reset)

% .setSrcs = LL_HRTIM_OUTPUTSET_TIMAEV5_TIMDCMP1 | LL_HRTIM_OUTPUTSET_EEV_9,
% .rstSrcs = LL_HRTIM_OUTPUTRESET_EEV_8,

persistent set_prev;
persistent reset_prev;
persistent ta2_prev;

% Init persistent var on first iter
if isempty(set_prev)
    set_prev = set; 
end

if isempty(reset_prev)
    reset_prev = reset; 
end

if isempty(ta2_prev)
    ta2_prev = 0; 
end

ta2 = ta2_prev;

% Check for rising edge on SET input
set_re  = (set > 0) && (set_prev <= 0); 
% Check for rising edge on RESET input
reset_re  = (reset > 0) && (reset_prev <= 0);

if set_re
    ta2 = 1;
end

if reset_re
    ta2 = 0;
end

% Update persistent var for next iteration
set_prev = set;
reset_prev = reset;
ta2_prev = ta2;

== matlab function HRTIM_main/TIMD: Pulse Skip/timd_td2 ==
  data: set input; td2 output; reset input
function td2 = timd_td2(set,reset)

persistent set_prev;
persistent reset_prev;
persistent td2_prev;

% Init persistent var on first iter
if isempty(set_prev)
    set_prev = set; 
end

if isempty(reset_prev)
    reset_prev = reset; 
end

if isempty(td2_prev)
    td2_prev = 0; 
end

td2 = td2_prev;

% Check for rising edge on SET input
set_re  = (set > 0) && (set_prev <= 0); 
% Check for rising edge on RESET input
reset_re  = (reset > 0) && (reset_prev <= 0);

if set_re
    td2 = 1;
end

if reset_re
    td2 = 0;
end


% Update persistent var for next iteration
set_prev = set;
reset_prev = reset;
td2_prev = td2;

== matlab function HRTIM_main/TIMF: Feedback Timeout Watchdog/timf_output ==
  data: set input; tf2 output; reset input
function tf2  = timf_tf2(set,reset)

persistent set_prev;
persistent reset_prev;
persistent tf2_prev;

% Init persistent var on first iter
if isempty(set_prev)
    set_prev = set; 
end

if isempty(reset_prev)
    reset_prev = reset; 
end


if isempty(tf2_prev)
    tf2_prev = 0; 
end

tf2 = tf2_prev;

% Check for rising edge on SET input
set_re  = (set > 0) && (set_prev <= 0); 
% Check for rising edge on RESET input
reset_re  = (reset > 0) && (reset_prev <= 0);

if set_re
    tf2 = 1;
end

if reset_re
    tf2 = 0;
end

% Update persistent var for next iteration
set_prev = set;
reset_prev = reset;
tf2_prev = tf2;

end

== matlab function HRTIM_main/TIMF: Feedback Timeout Watchdog/Capture TIMF.CPT2FR1 ==
  data: count input; cap output; trigger input; hit output
function [cap,hit] = capture_reg(count,trigger)

% hit generates positive pulse when capture occurs

persistent count_prev;
persistent trigger_prev;

persistent cap_reg;

% Init persistent variables
if isempty(count_prev)
    count_prev = count; 
end

if isempty(trigger_prev)
    trigger_prev = trigger; 
end

if isempty(cap_reg)
    cap_reg = uint16(0); 
end

hit = 0;

% Trigger rising edge detect
trigger_re  = (trigger > 0) && (trigger_prev <= 0); 

% Capture register on rising edge of trigger
% Use previous count since we are 1 sample behind
if trigger_re
    cap_reg = count_prev;
    hit = 1;
end

% Update persistent var
count_prev = count;
trigger_prev = trigger;

cap = cap_reg;
